simulink model "problem3b"  (R2026a)
settings: Solver=VariableStepAuto
values from neighbouring files (symbols this model uses):
  x = input(message)    [problem3bmatlab.m]
settings Model: Creator=rawad  LastModifiedBy=rawad

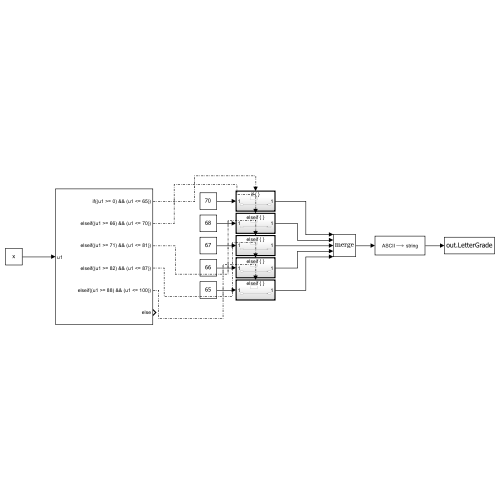
[thumbnail: Simulink's stored preview of the top-level diagram]
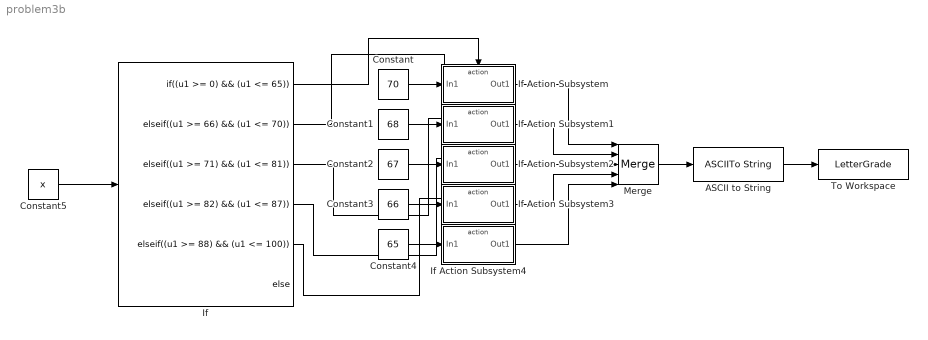
== system problem3b ==
  ASCII to String : ASCIIToString
  Constant : Constant  Value=70  OutDataTypeStr=uint8
  Constant1 : Constant  Value=68  OutDataTypeStr=uint8
  Constant2 : Constant  Value=67  OutDataTypeStr=uint8
  Constant3 : Constant  Value=66  OutDataTypeStr=uint8
  Constant4 : Constant  Value=65  OutDataTypeStr=uint8
  Constant5 : Constant  Value=x
  If : If  IfExpression=(u1 >= 0) && (u1 <= 65)  ElseIfExpressions=(u1 >= 66) && (u1 <= 70),(u1 >= 71) && (u1 <= 81),(u1 >= 82) && (u1 <= 87),(u1 >= 88) && (u1 <= 100)
  If Action Subsystem : Subsystem  TreatAsAtomicUnit=on
  If Action Subsystem1 : Subsystem  TreatAsAtomicUnit=on
  If Action Subsystem2 : Subsystem  TreatAsAtomicUnit=on
  If Action Subsystem3 : Subsystem  TreatAsAtomicUnit=on
  If Action Subsystem4 : Subsystem  TreatAsAtomicUnit=on
  Merge : Merge  Inputs=5
  To Workspace : ToWorkspace  VariableName=LetterGrade  SaveFormat=Timeseries  SampleTime=-1
  wires:
  If Action Subsystem/1(Out1) -> Merge/1
  If/3 -> If Action Subsystem2/Action
  Constant1/1 -> If Action Subsystem1/1(In1)
  If Action Subsystem4/1(Out1) -> Merge/5
  Constant4/1 -> If Action Subsystem4/1(In1)
  If/2 -> If Action Subsystem1/Action
  Constant2/1 -> If Action Subsystem2/1(In1)
  If/1 -> If Action Subsystem/Action
  Constant/1 -> If Action Subsystem/1(In1)
  If Action Subsystem1/1(Out1) -> Merge/2
  Merge/1 -> ASCII to String/1
  If Action Subsystem2/1(Out1) -> Merge/3
  If/4 -> If Action Subsystem3/Action
  Constant3/1 -> If Action Subsystem3/1(In1)
  If/5 -> If Action Subsystem4/Action
  If Action Subsystem3/1(Out1) -> Merge/4
  Constant5/1 -> If/1
  ASCII to String/1 -> To Workspace/1

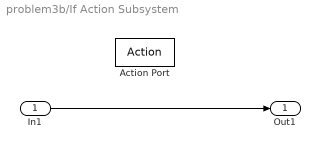
== system problem3b/If Action Subsystem ==
  In1 : Inport
  Action Port : ActionPort  ActionPortLabel=if((u1 >= 0) && (u1 <= 65))
  Out1 : Outport
  wires:
  In1/1 -> Out1/1

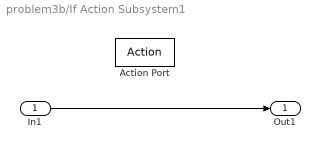
== system problem3b/If Action Subsystem1 ==
  In1 : Inport
  Action Port : ActionPort  ActionPortLabel=elseif((u1 >= 66) && (u1 <= 70))
  Out1 : Outport
  wires:
  In1/1 -> Out1/1

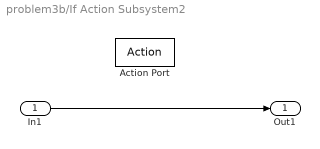
== system problem3b/If Action Subsystem2 ==
  In1 : Inport
  Action Port : ActionPort  ActionPortLabel=elseif((u1 >= 71) && (u1 <= 81))
  Out1 : Outport
  wires:
  In1/1 -> Out1/1

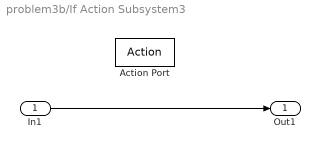
== system problem3b/If Action Subsystem3 ==
  In1 : Inport
  Action Port : ActionPort  ActionPortLabel=elseif((u1 >= 82) && (u1 <= 87))
  Out1 : Outport
  wires:
  In1/1 -> Out1/1

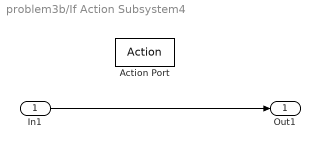
== system problem3b/If Action Subsystem4 ==
  In1 : Inport
  Action Port : ActionPort  ActionPortLabel=elseif((u1 >= 88) && (u1 <= 100))
  Out1 : Outport
  wires:
  In1/1 -> Out1/1
